simulink model "CIEControlSimulink"  (R2018b)
settings: Solver=FixedStepAuto  StartTime=0.0  StopTime=5  FixedStep=0.00005  MaxStep=0.001  MinStep=1e-3  RelTol=5e-3
PostLoadFcn:
  | helperLateralControlTutorialSetup
undefined symbols (not defined in the file or in its folder): animation_update_interval, datetime, directions, enable_CG_trace, enable_rearAxle_trace, plotAxisLimitMode, plotAxisLimits, refPoses, save_anim_frames, speedProfile, theta0, v0, vehicle_length, vehicle_width, wheelbase, x0, y0
libraries: autolibshared x1
settings Model: PacingRate=0.750000  Creator=The MathWorks, Inc.  LastModifiedBy=root
settings SolverCC: MaxConsecutiveMinStep=2  ZeroCrossAlgorithm=Adaptive  DecoupledContinuousIntegration=on  MinimalZcImpactIntegration=on
settings DataIOCC: SaveOutput=off  SignalLogging=off  DSMLogging=off  SaveTime=off
settings DebuggingCC: LibraryContextMissingDiagnostic=none
settings SFSimCC: SimUseLocalCustomCode=off
settings RTWCC: RTWUseLocalCustomCode=off

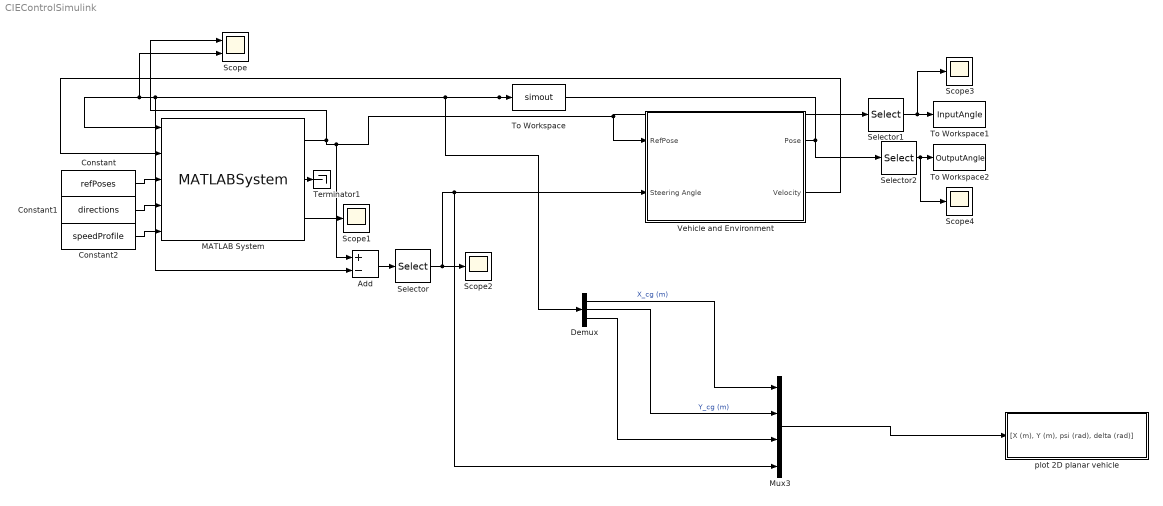
== system CIEControlSimulink ==
  Add : Sum  Inputs=+-
  Constant : Constant  Value=refPoses
  Constant1 : Constant  Value=directions
  Constant2 : Constant  Value=speedProfile
  Demux : Demux  Outputs=3
  MATLAB System : MATLABSystem  System=HelperPathAnalyzer  Wheelbase=wheelbase  HasResetOutput=off  SimulateUsing=Interpreted execution
      mask Type: HelperPathAnalyzer
      mask Display:
      | disp(['Helper' char(10) 'Path' char(10) 'Analyzer']);
      | port_label('input',1,'CurrPose');
      | port_label('input',2,'CurrVelocity');
      | port_label('input',3,'RefPoses');
      | port_label('input',4,'Directions');
      | port_label('input',5,'SpeedProfile');
      | port_label('output',1,'RefPose');
      | port_label('output',2,'RefVelocity');
      | port_label('output',3,'Direction');
  Mux3 : Mux
  Scope : Scope  NumInputPorts=2
  Scope{1..4} (4 alike) : Scope
  Selector : Selector  InputPortWidth=3  IndexOptions=Index vector (dialog)  Indices=[3]  OutputSizes=1
  Selector1 : Selector  InputPortWidth=3  IndexOptions=Index vector (dialog)  Indices=[3]  OutputSizes=1
  Selector2 : Selector  InputPortWidth=3  IndexOptions=Index vector (dialog)  Indices=[3]  OutputSizes=1
  Terminator1 : Terminator
  To Workspace : ToWorkspace  VariableName=simout  SampleTime=-1
  To Workspace1 : ToWorkspace  VariableName=InputAngle  SampleTime=-1
  To Workspace2 : ToWorkspace  VariableName=OutputAngle  SampleTime=-1
  Vehicle and Environment : Subsystem
  plot 2D planar vehicle : Subsystem  mask(6DoF Animation){axisMode=plotAxisLimitMode, ax=plotAxisLimits, Ts=animation_update_interval, enable_CG_trace=enable_CG_trace, enable_rearAxle_trace=enable_rearAxle_trace, save_anim_frames=save_anim_frames, anim_frame_name_str=char(datetime('now','Format','yyyy-MM-dd_HH_mm_ss')), L=vehicle_length, W=vehicle_width}
      mask prompts: axisMode "Axis Mode (0->auto, 1->fixed, BOTH use Axes Limits below)"; ax "Axes limits [xmin xmax ymin ymax] (m):"; Ts "Time interval between updates (s):"; enable_CG_trace "Enable vehicle CG trace? (0/1)"; enable_rearAxle_trace "Enable rear axle trace? (0/1)"; save_anim_frames "Save animaton frames? (0/1)"; anim_frame_name_str "Animation sequence name (if save frames==1)"; L "Vehicle length (m)"; W "Vehicle width (m)"
      mask help:
      | Create a 2D animated view of a steering vehicle model with tires.
      |
      | Marc Compere
      | CompereM@saic.com
      | created : 22 August 2002
      | modified: 28 Dec 2015
      mask init:
      | Config.axisMode=axisMode;
      | Config.ax=ax;
      | Config.Ts=Ts;
      | Config.enable_CG_trace=enable_CG_trace;
      | Config.enable_rearAxle_trace=enable_rearAxle_trace;
      | Config.save_anim_frames=save_anim_frames;
      | Config.anim_frame_name_str=anim_frame_name_str;
      | Config.L=L;
      | Config.W=W;
      mask Help:
      | <p>This block generates a 3 dimensional display of a simulation trajectory, with the craft orientation displayed during flight</p>
      | 
      | <p>There are two inputs to this block, Position and Euler.  These inputs contain more than one signal as described below.</p>
      | 
      | <p><H4>Block Vector Input - Position</H4>
      | <ul>
      | <li>X Position</li>
      | <li>Y Position</li>
      | <li>Z Position</li>
      | </ul>
      | </p>
      | 
      | <p><H4>Block Vector Input - Euler</H4>
      |     <ul>
      |     <li>Roll Attitude</li>
      |     <li>Pitch Attitude</li>
      |     <li>Yaw Attitude</li>
      |    </ul>
      |    </p>
  wires:
  Constant/1 -> MATLAB System/3
  MATLAB System/2 -> Terminator1/1
  MATLAB System/3 -> Scope1/1
  Constant2/1 -> MATLAB System/5
  Constant1/1 -> MATLAB System/4
  Vehicle and Environment/2(Velocity) -> MATLAB System/2
  MATLAB System/1 -> Selector1/1, Vehicle and Environment/1(RefPose), Add/1, Scope/1
  Add/1 -> Selector/1
  Selector1/1 -> Scope3/1, To Workspace1/1
  Selector2/1 -> Scope4/1, To Workspace2/1
  Demux/1 -> Mux3/1  "X_cg (m)"
  Demux/2 -> Mux3/2  "Y_cg (m)"
  Mux3/1 -> plot 2D planar vehicle/1("[X (m), Y (m), psi (rad), delta (rad)]")
  Selector/1 -> Mux3/4, Vehicle and Environment/2(Steering Angle), Scope2/1
  Vehicle and Environment/1(Pose) -> Selector2/1, Demux/1, Add/2, Scope/2, MATLAB System/1, To Workspace/1
  Demux/3 -> Mux3/3

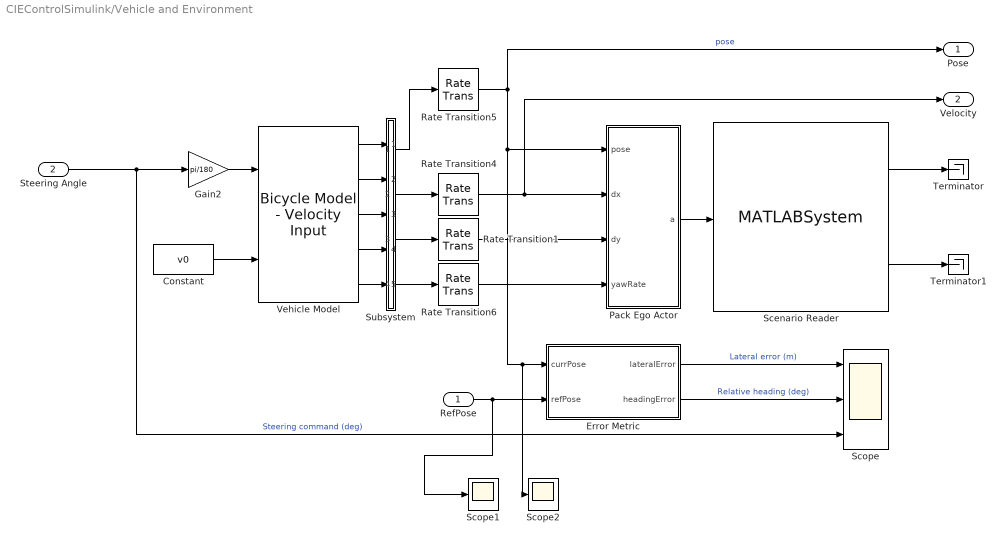
== system CIEControlSimulink/Vehicle and Environment ==
  RefPose : Inport
  Steering Angle : Inport  Port=2
  Constant : Constant  Value=v0
  Error Metric : MATLAB Function  TreatAsAtomicUnit=on  mask{wheelbase=wheelbase}
      mask prompts: wheelbase "Wheelbase of vehicle"
  Gain2 : Gain  Gain=pi/180
  Pack Ego Actor : MATLAB Function  TreatAsAtomicUnit=on
  Rate Transition1 : RateTransition  OutPortSampleTime=Ts
  Rate Transition4 : RateTransition  InitialCondition=v0  OutPortSampleTime=Ts
  Rate Transition5 : RateTransition  InitialCondition=[x0, y0, theta0]  OutPortSampleTime=Ts
  Rate Transition6 : RateTransition  OutPortSampleTime=Ts
  Scenario Reader : MATLABSystem  System=helperScenarioReader  ScenarioFileName=lateralControlTutorial  EgoActorSource=Input port  EgoActorID=1  RoadBoundaries=off  LaneBoundaries=off  AllBoundaries=off  LaneBoundaryDistance=0:0.5:60  LaneBoundaryLocation=inner  CurrentLane=off  NumLanes=off  LaneMarkings=on  BusNameSource=Auto  BusName2Source=Auto  BusName3Source=Auto  SimulateUsing=Interpreted execution
      mask Type: helperScenarioReader
      mask Display:
      | disp(['Scenario' char(10) 'Reader']);
      | port_label('input',1,'Ego Actor');
      | port_label('output',1,'Actors');
      | port_label('output',2,'Lane Markings');
  Scope : Scope  NumInputPorts=3
  Scope1 : Scope
  Scope2 : Scope
  Subsystem : Subsystem
  Terminator : Terminator
  Terminator1 : Terminator
  Vehicle Model : autolibshared/Bicycle Model - Velocity Input  trackMode=Single (bicycle)  inputMode=External longitudinal forces  frontSteerMode=on  rearSteerMode=off  windMode=off  muMode=off  extFMode=off  extMMode=off  aMode=3  NF=2  NR=2  m=2000  a=wheelbase/2  b=wheelbase/2  h=0.35  X_o=x0+cosd(theta0)*wheelbase/2  xdot_o=v0  CalphaMode=off  sigmaMode=on  w=[1.4,1.4]  Cy_f=12e3  Cy_r=11e3  sigma_f=.1  sigma_r=.1  alpha_f_brk=[-.1 .1]  Cy_f_data=[-9e3 9e3]  alpha_r_brk=[-.1 .1]  Cy_r_data=[-9e3 9e3]  Y_o=y0+sind(theta0)*wheelbase/2  ydot_o=0  Izz=4000  psi_o=deg2rad(theta0)  r_o=0  Af=2  Cd=.3  Cl=.1  Cpm=.1  beta_w=[0:0.01:0.3]  Cs=[0:0.03:0.9]  Cym=[0:0.01:0.3]  Pabs=101325  Tair=273  g=9.81  mu=1  xdot_tol=0.01  Fznom=5000  Fxtire_sat=1e6  Fytire_sat=1e6  longOff=0  latOff=0  vertOff=0
      settings: SourceProductName=Powertrain Blockset  SourceProductBaseCode=PW
  Pose : Outport
  Velocity : Outport  Port=2
  wires:
  Rate Transition4/1 -> Pack Ego Actor/2(dx), Velocity/1
  Subsystem/3(Out3) -> Rate Transition1/1
  Subsystem/2(Out2) -> Rate Transition4/1
  Subsystem/1(Out1) -> Rate Transition5/1
  Rate Transition6/1 -> Pack Ego Actor/4(yawRate)
  Subsystem/4(Out4) -> Rate Transition6/1
  Scenario Reader/1 -> Terminator/1
  Rate Transition1/1 -> Pack Ego Actor/3(dy)
  Pack Ego Actor/1(a) -> Scenario Reader/1
  Scenario Reader/2 -> Terminator1/1
  Rate Transition5/1 -> Scope2/1, Error Metric/1(currPose), Pack Ego Actor/1(pose), Pose/1  "pose"
  Error Metric/1(lateralError) -> Scope/1  "Lateral error (m)"
  RefPose/1 -> Scope1/1, Error Metric/2(refPose)
  Steering Angle/1 -> Scope/3, Gain2/1  "Steering command (deg)"
  Error Metric/2(headingError) -> Scope/2  "Relative heading (deg)"
  Gain2/1 -> Vehicle Model/1
  Constant/1 -> Vehicle Model/2
  Vehicle Model/4 -> Subsystem/4(In4)
  Vehicle Model/5 -> Subsystem/5(In5)
  Vehicle Model/1 -> Subsystem/1(In1)
  Vehicle Model/2 -> Subsystem/2(In2)
  Vehicle Model/3 -> Subsystem/3(In3)

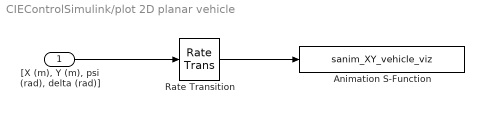
== system CIEControlSimulink/plot 2D planar vehicle ==
  "[X (m), Y (m), psi (rad), delta (rad)]" : Inport
  Animation S-Function : S-Function  FunctionName=sanim_XY_vehicle_viz  Parameters=Config  SFunctionDeploymentMode=off  EnableBusSupport=off
  Rate Transition : RateTransition  Integrity=off
  wires:
  "[X (m), Y (m), psi (rad), delta (rad)]"/1 -> Rate Transition/1
  Rate Transition/1 -> Animation S-Function/1

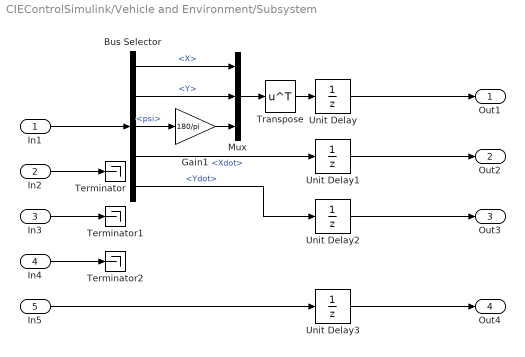
== system CIEControlSimulink/Vehicle and Environment/Subsystem ==
  In1 : Inport
  In2 : Inport  Port=2
  In3 : Inport  Port=3
  In4 : Inport  Port=4
  In5 : Inport  Port=5
  Bus Selector : BusSelector  OutputSignals=InertFrm.RearAxl.Disp.X,InertFrm.RearAxl.Disp.Y,InertFrm.Cg.Ang.psi,InertFrm.RearAxl.Vel.Xdot,InertFrm.RearAxl.Vel.Ydot
  Gain1 : Gain  Gain=180/pi
  Mux : Mux  Inputs=3
  Terminator : Terminator
  Terminator1 : Terminator
  Terminator2 : Terminator
  Transpose : Math  Operator=transpose  SaturateOnIntegerOverflow=on
  Unit Delay : UnitDelay  InitialCondition=[x0, y0, theta0]  SampleTime=-1
  Unit Delay1 : UnitDelay  InitialCondition=v0  SampleTime=-1
  Unit Delay2 : UnitDelay  SampleTime=-1
  Unit Delay3 : UnitDelay  SampleTime=-1
  Out1 : Outport
  Out2 : Outport  Port=2
  Out3 : Outport  Port=3
  Out4 : Outport  Port=4
  wires:
  Bus Selector/4 -> Unit Delay1/1  "<Xdot>"
  Bus Selector/2 -> Mux/2  "<Y>"
  Bus Selector/1 -> Mux/1  "<X>"
  Transpose/1 -> Unit Delay/1
  Unit Delay/1 -> Out1/1
  Mux/1 -> Transpose/1
  Unit Delay3/1 -> Out4/1
  Bus Selector/5 -> Unit Delay2/1  "<Ydot>"
  Bus Selector/3 -> Gain1/1  "<psi>"
  Gain1/1 -> Mux/3
  In5/1 -> Unit Delay3/1
  In2/1 -> Terminator/1
  In1/1 -> Bus Selector/1
  In4/1 -> Terminator2/1
  Unit Delay2/1 -> Out3/1
  Unit Delay1/1 -> Out2/1
  In3/1 -> Terminator1/1

== matlab function CIEControlSimulink/Vehicle and Environment/Error Metric ==
  data: currPose input size=[1 3]; refPose input size=[1 3]; lateralError output; wheelbase parameter; headingError output
function [lateralError, headingError] = fcn(currPose, refPose, wheelbase)

%   Copyright 2018 The MathWorks, Inc.

currPose(:,3) = deg2rad(currPose(:,3));
refPose(:,3)  = deg2rad(refPose(:,3));

%Convert current pose to front wheel coordinate
currPoseF = coder.nullcopy(zeros(1, 3));

currPoseF = driving.internal.control.rearPoseToFrontPose(currPose, wheelbase);

lateralError = norm(currPoseF(1:2) - refPose(1:2));

headingError = rad2deg(currPose(:, 3) - refPose(:,3));

== matlab function CIEControlSimulink/Vehicle and Environment/Pack Ego Actor ==
  data: pose input; a output Bus: BusActors1Actors size=1; dx input; dy input; yawRate input
function a = packEgo(pose,dx,dy,yawRate)
% Pack ego information into a single ego actor bus
%
% Imoprtant note:
% Output is a bus of type BusActorsActors. This is the same bus used by the
% helperScenarioReader to output an individual actor. If you change the
% output bus name of helperScenarioReader, change the output bus name here
% as well by clicking on 'Edit Data' in the menu above.

a = struct(...
    'ActorID',1,...
    'Position', [pose(1) pose(2) 0], ...
    'Velocity', [dx dy 0], ...
    'Roll', 0, ...
    'Pitch', 0, ...
    'Yaw', pose(3), ...
    'AngularVelocity', [0 0 yawRate]);
